simulink model "LunarMicrogrid_Full_Arch"  (R2026b)
settings: Solver=ode23t  StopTime=simulation.timeSim  MaxStep=1/(5*solarPlant.converterSwitchingFrequency)  AbsTol=1e-3
PreLoadFcn:
  | run('LunarMicrogridA_Data');
values from neighbouring files (symbols this model uses):
  Csc = Csc_cell/Ns_sc*Np_sc    (= 200)    [LunarDAB_Params.m]
  eta_sc = 0.95    [LunarDAB_Params.m]
  fsw = 100e3    (= 100000)    [LunarDAB_Params.m]
  k_restore = 1    [LunarDAB_Params.m]
  kiCurrent = 2    [LunarDAB_Params.m]
  kiVoltage = 8    [LunarDAB_Params.m]
  kpCurrent = 0.005    [LunarDAB_Params.m]
  kpVoltage = 0.4    [LunarDAB_Params.m]
  lTotal = lSeries + Llk    [LunarDAB_Params.m]
  P170_dt = 1e-4    (= 0.0001)    [P170_PV_Initialize.m]
  P170_Imp = im(ix)    [P170_PV_Initialize.m]
  P170_Vmp = vm(ix)    [P170_PV_Initialize.m]
  Rd_bat = dV_droop/Ibat_max    (= 0.232258064516)    [LunarDAB_Params.m]
  SC_enable = 1    [LunarDAB_Params.m]
  thetaIC = 0    [LunarDAB_Params.m]
  thetaMaxDab = pi/4    (= 0.785398163397)    [LunarDAB_Params.m]
  Tsw = 1/fsw    (= 1e-05)    [LunarDAB_Params.m]
  Vsc0 = sqrt((Vsc_max^2 + Vsc_min^2)/2)    [LunarDAB_Params.m]
  Vsc_max = 119    [LunarDAB_Params.m]
  Vsc_min = 66    [LunarDAB_Params.m]
undefined symbols (not defined in the file or in its folder): a_lpf_sys, battery, bms, connectedLoad, dcVoltage, DiscIntNeverNeededParam, eta_dab, Ibat_sign, mmc, Ndab, P170_T, pvDroop, sc, sensor, socLimit, solarPlant
libraries: sl_discontinuities x13, fl_lib x13, nesl_utility x13, simulink x7, batteryecm_lib x1, simulink_extras x1, ee_lib x1
(part 4 of 8)

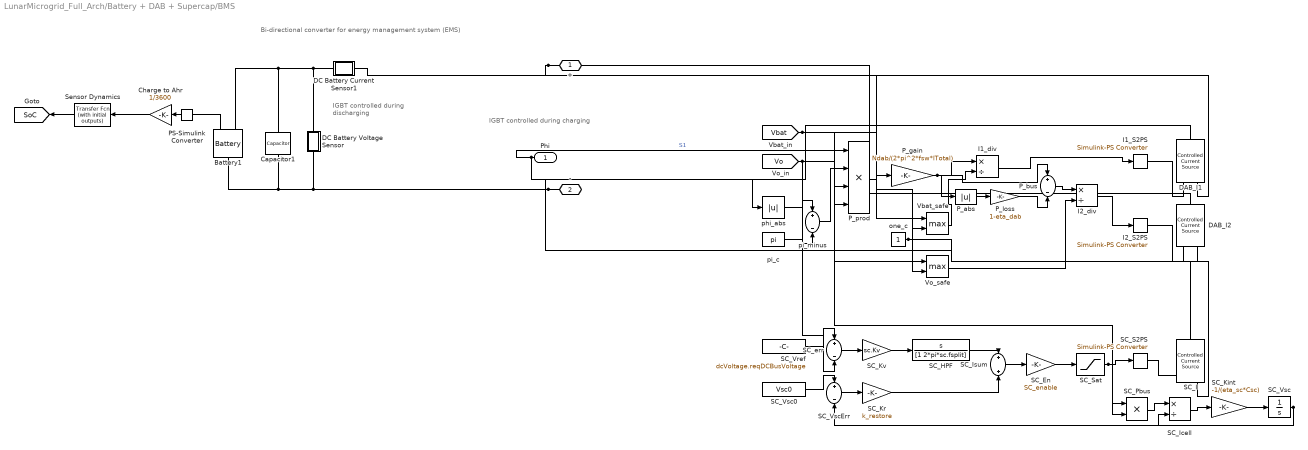
== system LunarMicrogrid_Full_Arch/Battery + DAB + Supercap/BMS ==
  note: IGBT controlled during charging
  note: Bi-directional converter for energy management system (EMS)
  note: IGBT controlled during discharging
  Phi : Inport
  Battery1 : batteryecm_lib/Battery  Vnom=battery.nominalBatteryVoltage V  prm_dir=1  R1_dis=2 Ohm  R1_ch=2 Ohm  R1=0.01 Ohm  prm_AH=2  AH=connectedLoad.batteryAmpHr hr*A  V1=battery.minBatteryNominalVoltage V  AH1=connectedLoad.batteryAmpHr*0.2 hr*A  prm_R2=2  R2=2000 Ohm  Tmeas=298.15 K  charge_measurement_port=simscape.enum.battery.enable.yes  prm_dyn=1  Rp1=0.005 Ohm  tau1=30 s  Rp2=0.005 Ohm  tau2=30 s  Rp3=0.005 Ohm  tau3=30 s  Rp4=0.005 Ohm  tau4=30 s  Rp5=0.005 Ohm  tau5=30 s  prm_fade=1  N_fade=100  AH_fade=45 hr*A  R1_fade=2.02 Ohm  R1_ch_fade=2.02 Ohm  V1_fade=10.35 V  prm_age=1  prm_age_OCV=1  OCV_age=0.9  SOC_age=60  Tmeas_age=298.15 K  delta_time_age_vec=[0] d  temperature_age_vec=[273] K  OCV_scaling_age=2.2134e6  OCV_offset_age=1.632e6  temp_exp_age=0.515833569 V  t_exp_age=0.75  Vnom_T2=12 V  R1_T2=2.2 Ohm  R1_T2_dis=2.2 Ohm  R1_T2_ch=2.2 Ohm  V1_T2=11.4 V  R2_T2=2200 Ohm  Rp1_T2=0.005 Ohm  tau1_T2=30 s  Rp2_T2=0.005 Ohm  tau2_T2=30 s  Rp3_T2=0.005 Ohm  tau3_T2=30 s  Rp4_T2=0.005 Ohm  tau4_T2=30 s  Rp5_T2=0.005 Ohm  tau5_T2=30 s  Tmeas2=273.15 K  thermal_port=simscape.enum.thermaleffects.omit  thermal_mass=30000 J/K  i_specify=off  i_priority=None  i=0 A  i_nominal_specify=off  i_nominal_value=1  i_nominal_unit=A  v_specify=off  v_priority=None  v=0 V  v_nominal_specify=off  v_nominal_value=1  v_nominal_unit=V  charge_specify=on  charge_priority=High  charge=batteryInitialStateOfCharge hr*A  charge_nominal_specify=off  charge_nominal_value=1  charge_nominal_unit=A*hr  num_cycles_specify=off  num_cycles_priority=High  num_cycles=0  num_cycles_nominal_specify=off  num_cycles_nominal_value=1  num_cycles_nominal_unit=1  temperature_specify=off  temperature_priority=High  temperature=298.15 K  temperature_nominal_specify=off  temperature_nominal_value=1  temperature_nominal_unit=K
  Capacitor1 : fl_lib/Electrical/Electrical Elements/Capacitor  c=boost.outputCapacitor F  r=1e-6 Ohm  g=0 1/Ohm  i_specify=off  i_priority=None  i=0 A  i_nominal_specify=off  i_nominal_value=1  i_nominal_unit=A  v_specify=off  v_priority=None  v=0 V  v_nominal_specify=off  v_nominal_value=1  v_nominal_unit=V  vc_specify=on  vc_priority=High  vc=batteryInputCapacitorInitialVoltage V  vc_nominal_specify=off  vc_nominal_value=1  vc_nominal_unit=V
  Charge to Ahr : Gain  Gain=1/3600
  DAB_I1 : fl_lib/Electrical/Electrical Sources/Controlled Current Source
  DAB_I2 : fl_lib/Electrical/Electrical Sources/Controlled Current Source
  DC Battery Current Sensor1 : Subsystem
      mask Display: disp('i');
  DC Battery Voltage Sensor : Subsystem
      mask Display: disp('v');
  I1_S2PS : nesl_utility/Simulink-PS Converter  PhysicalDomain=network_engine_domain  SubClassName=ps_input  LeftPortType=input  RightPortType=output  PseudoPeriodic=off  Frequencies=[]  NoiseDistribution=none  NoiseParameters=[]  Unit=1  AffineConversion=off  FilteringAndDerivatives=provide  SimscapeFilterOrder=1  InputFilterTimeConstant=0.001  UdotUserProvided=0
  I1_div : Product  Inputs=*/
  I2_S2PS : nesl_utility/Simulink-PS Converter  PhysicalDomain=network_engine_domain  SubClassName=ps_input  LeftPortType=input  RightPortType=output  PseudoPeriodic=off  Frequencies=[]  NoiseDistribution=none  NoiseParameters=[]  Unit=1  AffineConversion=off  FilteringAndDerivatives=provide  SimscapeFilterOrder=1  InputFilterTimeConstant=0.001  UdotUserProvided=0
  I2_div : Product  Inputs=*/
  PS-Simulink Converter : nesl_utility/PS-Simulink Converter  PhysicalDomain=network_engine_domain  SubClassName=ps_output  LeftPortType=input  RightPortType=output  PseudoPeriodic=off  Frequencies=[]  VectorFormat=1-D array  Unit=inherit  AffineConversion=off
  P_abs : Abs  SaturateOnIntegerOverflow=off
  P_bus : Sum  Inputs=+-
  P_gain : Gain  Gain=Ndab/(2*pi^2*fsw*lTotal)
  P_loss : Gain  Gain=1-eta_dab
  P_prod : Product  Inputs=4
  SC_En : Gain  Gain=SC_enable
  SC_HPF : TransferFcn  Numerator=[1 0]  Denominator=[1 2*pi*sc.fsplit]
  SC_I : fl_lib/Electrical/Electrical Sources/Controlled Current Source
  SC_Icell : Product  Inputs=*/
  SC_Isum : Sum
  SC_Kint : Gain  Gain=-1/(eta_sc*Csc)
  SC_Kr : Gain  Gain=k_restore
  SC_Kv : Gain  Gain=sc.Kv
  SC_Pbus : Product
  SC_S2PS : nesl_utility/Simulink-PS Converter  PhysicalDomain=network_engine_domain  SubClassName=ps_input  LeftPortType=input  RightPortType=output  PseudoPeriodic=off  Frequencies=[]  NoiseDistribution=none  NoiseParameters=[]  Unit=1  AffineConversion=off  FilteringAndDerivatives=provide  SimscapeFilterOrder=1  InputFilterTimeConstant=0.001  UdotUserProvided=0
  SC_Sat : Saturate  UpperLimit=sc.Imax  LowerLimit=-sc.Imax
  SC_Vref : Constant  Value=dcVoltage.reqDCBusVoltage
  SC_Vsc : Integrator  InitialCondition=Vsc0  LimitOutput=on  UpperSaturationLimit=Vsc_max  LowerSaturationLimit=Vsc_min
  SC_Vsc0 : Constant  Value=Vsc0
  SC_VscErr : Sum  Inputs=+-
  SC_err : Sum  Inputs=+-
  Sensor Dynamics : simulink_extras/Additional Linear/Transfer Fcn (with initial outputs)  N=[1]  D=[1/sensor.samplingFreq 1]  Y0=batteryInitialStateOfCharge  U0=0
  Vbat_safe : MinMax  Function=max  Inputs=2
  Vo_safe : MinMax  Function=max  Inputs=2
  one_c : Constant
  phi_abs : Abs  SaturateOnIntegerOverflow=off
  pi_c : Constant  Value=pi
  pi_minus : Sum  Inputs=+-
  + : PMIOPort  Side=Right
  - : PMIOPort  Port=2  Side=Right
  tag scope: SoC=global
  wires:
  PS-Simulink Converter/1 -> Charge to Ahr/1
  Sensor Dynamics/1 -> [SoC]
  Charge to Ahr/1 -> Sensor Dynamics/1
  Phi/1 -> phi_abs/1, P_prod/1  "S1"
  pi_c/1 -> pi_minus/1
  phi_abs/1 -> pi_minus/2
  pi_minus/1 -> P_prod/2
  [Vbat] -> P_prod/3, Vbat_safe/1
  [Vo] -> P_prod/4, Vo_safe/1, SC_err/2, SC_Pbus/2
  P_prod/1 -> P_gain/1
  one_c/1 -> Vbat_safe/2, Vo_safe/2
  P_gain/1 -> I1_div/1, P_abs/1, P_bus/1
  Vbat_safe/1 -> I1_div/2
  P_abs/1 -> P_loss/1
  P_loss/1 -> P_bus/2
  P_bus/1 -> I2_div/1
  Vo_safe/1 -> I2_div/2
  SC_Vref/1 -> SC_err/1
  SC_err/1 -> SC_Kv/1
  SC_Kv/1 -> SC_HPF/1
  SC_Vsc0/1 -> SC_VscErr/1
  SC_Vsc/1 -> SC_VscErr/2, SC_Icell/2
  SC_VscErr/1 -> SC_Kr/1
  SC_HPF/1 -> SC_Isum/1
  SC_Kr/1 -> SC_Isum/2
  SC_Isum/1 -> SC_En/1
  SC_En/1 -> SC_Sat/1
  SC_Sat/1 -> SC_Pbus/1, SC_S2PS/1
  SC_Pbus/1 -> SC_Icell/1
  SC_Icell/1 -> SC_Kint/1
  SC_Kint/1 -> SC_Vsc/1
  I1_div/1 -> I1_S2PS/1
  I2_div/1 -> I2_S2PS/1
  connections:
  Battery1/RConn1 -- Capacitor1/RConn1 -- DC Battery Voltage Sensor/LConn1 -- DAB_I1/LConn1 -- DAB_I2/RConn2 -- -/RConn1 -- SC_I/RConn2
  Battery1/LConn2 -- PS-Simulink Converter/LConn1
  DC Battery Current Sensor1/LConn1 -- DC Battery Voltage Sensor/RConn1 -- Battery1/LConn1 -- Capacitor1/LConn1
  I1_S2PS/RConn1 -- DAB_I1/RConn1
  I2_S2PS/RConn1 -- DAB_I2/RConn1
  SC_S2PS/RConn1 -- SC_I/RConn1
  DAB_I1/RConn2 -- DC Battery Current Sensor1/RConn1
  +/RConn1 -- DAB_I2/LConn1 -- SC_I/LConn1

== system LunarMicrogrid_Full_Arch/Load (Site A)/Load ==
  AC Current Sensor2 : Subsystem
      mask Display: disp('i');
  Load : Subsystem
  Load Flag : Subsystem
  Load Resistance : fl_lib/Electrical/Electrical Elements/Variable Resistor  Rmin=0 Ohm  thermalEnable=false  thermal_mass=1 J/K  i_specify=off  i_priority=None  i=5 A  i_nominal_specify=off  i_nominal_value=1  i_nominal_unit=A  v_specify=off  v_priority=None  v=0 V  v_nominal_specify=off  v_nominal_value=1  v_nominal_unit=V  T_specify=off  T_priority=None  T=300 K  T_nominal_specify=off  T_nominal_value=1  T_nominal_unit=K
  SPST Switch : ee_lib/Switches & Breakers/SPST Switch  R_closed=0.01 Ohm  G_open=1e-6 S  Threshold=0.5 V  Width=0 V  model_dynamics=0  t_on=1e-3 s  t_off=1e-3 s  initial_vT=0 V
  + : PMIOPort  Side=Left
  - : PMIOPort  Port=2  Side=Right
  connections:
  +/RConn1 -- SPST Switch/LConn2
  Load Resistance/LConn2 -- AC Current Sensor2/LConn1
  Load Resistance/RConn1 -- -/RConn1
  Load/RConn1 -- Load Resistance/LConn1
  Load Flag/RConn1 -- SPST Switch/LConn1
  AC Current Sensor2/RConn1 -- SPST Switch/RConn1

== system LunarMicrogrid_Full_Arch/Low Voltage Bus (120 V)/DC Output Voltage Sensor ==
  PS-Simulink Converter : nesl_utility/PS-Simulink Converter  PhysicalDomain=network_engine_domain  SubClassName=ps_output  LeftPortType=input  RightPortType=output  PseudoPeriodic=off  Frequencies=[]  VectorFormat=1-D array  Unit=1  AffineConversion=off
  Sensor dynamics : TransferFcn  Numerator=1  Denominator=[1/sensor.samplingFreq 1]
  Voltage Sensor : fl_lib/Electrical/Electrical Sensors/Voltage Sensor
  - : PMIOPort  Side=Left
  + : PMIOPort  Port=2  Side=Right
  tag scope: Vo=global
  wires:
  PS-Simulink Converter/1 -> Sensor dynamics/1
  Sensor dynamics/1 -> [Vo]
  connections:
  Voltage Sensor/RConn2 -- -/RConn1
  Voltage Sensor/RConn1 -- PS-Simulink Converter/LConn1
  Voltage Sensor/LConn1 -- +/RConn1

== system LunarMicrogrid_Full_Arch/Monitoring/PV System Monitoring Panel ==
  note: Red - Overload , reduce the load and manually toggle the switch to restart the system
  note: Solar PV System Monitoring Panel
  note: Simulation time:
      | Increase the value for 'simulation.timeSim' to simulate for longer when exploring mode changes.
  note: Inputs:
      | Use the rotary controls to change the irradiance and load resistance during simulation.
  note: System overload (Mode-6):
      | System overload is triggered 'olTime' sec after the overload event. This delay is to ensure that it is not triggered because of transients. Parameter 'olTime' can be modified in the supporting livescript.
  note: Efficiency:
      | Percent efficiency may exceed 100% due to the stored energy in the inductor and capacitor. Efficiency value will be accurate in steady state.
  note: Battery sign convention:
      | +ve value for charging
      | -ve value for discharging
  Display{,1..6} (7 alike) : DisplayBlock  Transparency=1  GridColor=[0.502, 0.502, 0.502]
  Half Gauge : SemiCircularGaugeBlock  ScaleMin=20  FontColor=[0.0, 0.0, 0.0]
  Half Gauge1 : SemiCircularGaugeBlock  FontColor=[0.0, 0.0, 0.0]
  Lamp : LampBlock  DefaultColor=[192.0, 192.0, 192.0]
  Linear Gauge : LinearGaugeBlock  ScaleMin=-100  FontColor=[0.0, 0.0, 0.0]
  Monitoring : Subsystem
  PV MPPT Battery Charge Load ShutDown : LampBlock  DefaultColor=[192.0, 192.0, 192.0]
  PV MPPT Battery Discharge : LampBlock  DefaultColor=[192.0, 192.0, 192.0]
  PV MPPT Battery charge : LampBlock  DefaultColor=[192.0, 192.0, 192.0]
  PV ShutDown Battery Discharge : LampBlock  DefaultColor=[192.0, 192.0, 192.0]
  PV ShutDown Battery Isolated System ShutDown : LampBlock  DefaultColor=[192.0, 192.0, 192.0]
  PV Volt Control Battery Isolated : LampBlock  DefaultColor=[192.0, 192.0, 192.0]
  Start Mode : LampBlock  DefaultColor=[192.0, 192.0, 192.0]
  Toggle Switch1 : ToggleSwitchBlock

== system LunarMicrogrid_Full_Arch/PV Array + Converter/Irradiance ==
  Goto11 : Terminator
  Profile : FromWorkspace  VariableName=G_sim  Interpolate=off  OutputAfterFinalValue=Holding final value
  Sensor dynamics : TransferFcn  Numerator=1  Denominator=[1/sensor.samplingFreq 1]
  Solar Irradiance W/m2 : Gain
  Irad : Outport
  wires:
  Solar Irradiance W/m2/1 -> Irad/1, Sensor dynamics/1
  Profile/1 -> Solar Irradiance W/m2/1
  Sensor dynamics/1 -> Goto11/1

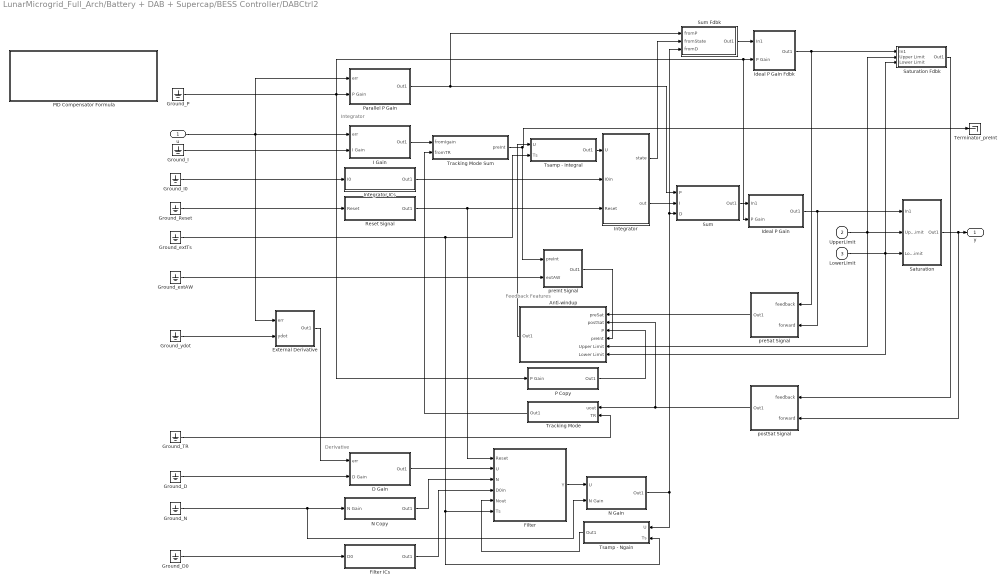
== system LunarMicrogrid_Full_Arch/Battery + DAB + Supercap/BESS Controller/DABCtrl2 ==
  note: Feedback Features
  note: Derivative
  note: Integrator
  u : Inport  SampleTime=SampleTime
  UpperLimit : Inport  Port=2
  LowerLimit : Inport  Port=3
  Anti-windup : Subsystem  Variant=on  VariantControlMode=label  VariantControl=Variant1  LabelModeActiveChoice=DiscClampingParallel
  D Gain : Subsystem  Variant=on  VariantControlMode=label  VariantControl=Variant1  LabelModeActiveChoice=Disabled
  External Derivative : Subsystem  Variant=on  VariantControlMode=label  VariantControl=Variant1  LabelModeActiveChoice=Disabled
  Filter : Subsystem  Variant=on  VariantControlMode=label  LabelModeActiveChoice=Disabled
  Filter ICs : Subsystem  Variant=on  VariantControlMode=label  VariantControl=Variant1  LabelModeActiveChoice=Disabled
  Ground_D : Ground
  Ground_D0 : Ground
  Ground_I : Ground
  Ground_I0 : Ground
  Ground_N : Ground
  Ground_P : Ground
  Ground_Reset : Ground
  Ground_TR : Ground  DisableCoverage=on
  Ground_extAW : Ground
  Ground_extTs : Ground
  Ground_ydot : Ground
  I Gain : Subsystem  Variant=on  VariantControlMode=label  VariantControl=Variant1  LabelModeActiveChoice=InternalParameters
  Ideal P Gain : Subsystem  Variant=on  VariantControlMode=label  VariantControl=Variant1  LabelModeActiveChoice=Disabled
  Ideal P Gain Fdbk : Subsystem  Variant=on  VariantControlMode=label  VariantControl=Variant1  LabelModeActiveChoice=Disabled
  Integrator : Subsystem  Variant=on  VariantControlMode=label  LabelModeActiveChoice=Discrete
  Integrator ICs : Subsystem  Variant=on  VariantControlMode=label  VariantControl=Variant1  LabelModeActiveChoice=InternalICs
  N Copy : Subsystem  Variant=on  VariantControlMode=label  LabelModeActiveChoice=Disabled_SignalSpec
  N Gain : Subsystem  Variant=on  VariantControlMode=label  VariantControl=Variant1  LabelModeActiveChoice=Disabled
  P Copy : Subsystem  Variant=on  VariantControlMode=label  LabelModeActiveChoice=Disabled
  PID Compensator Formula : Subsystem
      mask Display: image('/MATLAB/toolbox/simulink/library/pid/pid_Images/PI_Parallel_DT_0.png','center');
  Parallel P Gain : Subsystem  Variant=on  VariantControlMode=label  VariantControl=Variant1  LabelModeActiveChoice=InternalParameters
  Reset Signal : Subsystem  Variant=on  VariantControlMode=label  VariantControl=Variant1  LabelModeActiveChoice=Disabled
  Saturation : Subsystem  Variant=on  VariantControlMode=label  LabelModeActiveChoice=External
  Saturation Fdbk : Subsystem  Variant=on  VariantControlMode=label  LabelModeActiveChoice=Disabled
  Sum : Subsystem  Variant=on  VariantControlMode=label  LabelModeActiveChoice=Sum_PI
  Sum Fdbk : Subsystem  DisableCoverage=on  Variant=on  VariantControlMode=label  LabelModeActiveChoice=Disabled
  Terminator_preInt : Terminator
  Tracking Mode : Subsystem  Variant=on  VariantControlMode=label  VariantControl=Variant1  LabelModeActiveChoice=Disabled
  Tracking Mode Sum : Subsystem  Variant=on  VariantControlMode=label  LabelModeActiveChoice=Passthrough
  Tsamp - Integral : Subsystem  Variant=on  VariantControlMode=label  LabelModeActiveChoice=Disabled_SignalSpec
  Tsamp - Ngain : Subsystem  Variant=on  VariantControlMode=label  LabelModeActiveChoice=Passthrough
  postSat Signal : Subsystem  Variant=on  VariantControlMode=label  VariantControl=Variant1  LabelModeActiveChoice=Forward
  preInt Signal : Subsystem  Variant=on  VariantControlMode=label  VariantControl=Variant1  LabelModeActiveChoice=InternalPreInt
  preSat Signal : Subsystem  Variant=on  VariantControlMode=label  VariantControl=Variant1  LabelModeActiveChoice=Forward
  y : Outport  SampleTime=SampleTime
  wires:
  Ground_extAW/1 -> preInt Signal/2(extAW)
  preInt Signal/1(Out1) -> Anti-windup/4(preInt)
  External Derivative/1(Out1) -> D Gain/1(err)
  Ground_ydot/1 -> External Derivative/2(ydot)
  LowerLimit/1 -> Saturation/3(Lower Limit), Anti-windup/6(Lower Limit), Saturation Fdbk/3(Lower Limit)
  UpperLimit/1 -> Saturation/2(Upper Limit), Saturation Fdbk/2(Upper Limit), Anti-windup/5(Upper Limit)
  Tsamp - Ngain/1(Out1) -> Filter/5(Nout)
  Anti-windup/1(Out1) -> Tsamp - Integral/1(U)
  Ground_extTs/1 -> Tsamp - Integral/2(Ts), Filter/6(Ts), Tsamp - Ngain/2(Ts)
  Tsamp - Integral/1(Out1) -> Integrator/1(U)
  Tracking Mode/1(Out1) -> Tracking Mode Sum/2(fromTR)
  Ground_I0/1 -> Integrator ICs/1(I0)
  Filter ICs/1(Out1) -> Filter/4(D0in)
  N Copy/1(Out1) -> Filter/3(N)
  D Gain/1(Out1) -> Filter/2(U)
  Ground_D0/1 -> Filter ICs/1(D0)
  Ground_Reset/1 -> Reset Signal/1(Reset)
  N Gain/1(Out1) -> Tsamp - Ngain/1(U), Sum/3(D), Sum Fdbk/3(fromD)
  postSat Signal/1(Out1) -> Anti-windup/2(postSat), Tracking Mode/1(uout)
  preSat Signal/1(Out1) -> Anti-windup/1(preSat)
  Saturation Fdbk/1(Out1) -> postSat Signal/1(feedback)
  P Copy/1(Out1) -> Anti-windup/3(P)
  Ground_TR/1 -> Tracking Mode/2(TR)
  Ground_N/1 -> N Copy/1(N Gain), N Gain/2(N Gain)
  Ideal P Gain Fdbk/1(Out1) -> preSat Signal/1(feedback), Saturation Fdbk/1(In1)
  Sum Fdbk/1(Out1) -> Ideal P Gain Fdbk/1(In1)
  I Gain/1(Out1) -> Tracking Mode Sum/1(fromIgain)
  Saturation/1(Out1) -> y/1, postSat Signal/2(forward)
  Filter/1(Y) -> N Gain/1(U)
  Ground_D/1 -> D Gain/2(D Gain)
  Ideal P Gain/1(Out1) -> Saturation/1(In1), preSat Signal/2(forward)
  u/1 -> External Derivative/1(err), Parallel P Gain/1(err), I Gain/1(err)
  Parallel P Gain/1(Out1) -> Sum/1(P), Sum Fdbk/1(fromP)
  Sum/1(Out1) -> Ideal P Gain/1(In1)
  Ground_P/1 -> Ideal P Gain Fdbk/2(P Gain), Ideal P Gain/2(P Gain), Parallel P Gain/2(P Gain), P Copy/1(P Gain)
  Tracking Mode Sum/1(preInt) -> Terminator_preInt/1, preInt Signal/1(preInt)
  Ground_I/1 -> I Gain/2(I Gain)
  Integrator ICs/1(Out1) -> Integrator/2(I0in)
  Integrator/2(out) -> Sum/2(I)
  Integrator/1(state) -> Sum Fdbk/2(fromState)
  Reset Signal/1(Out1) -> Filter/1(Reset), Integrator/3(Reset)

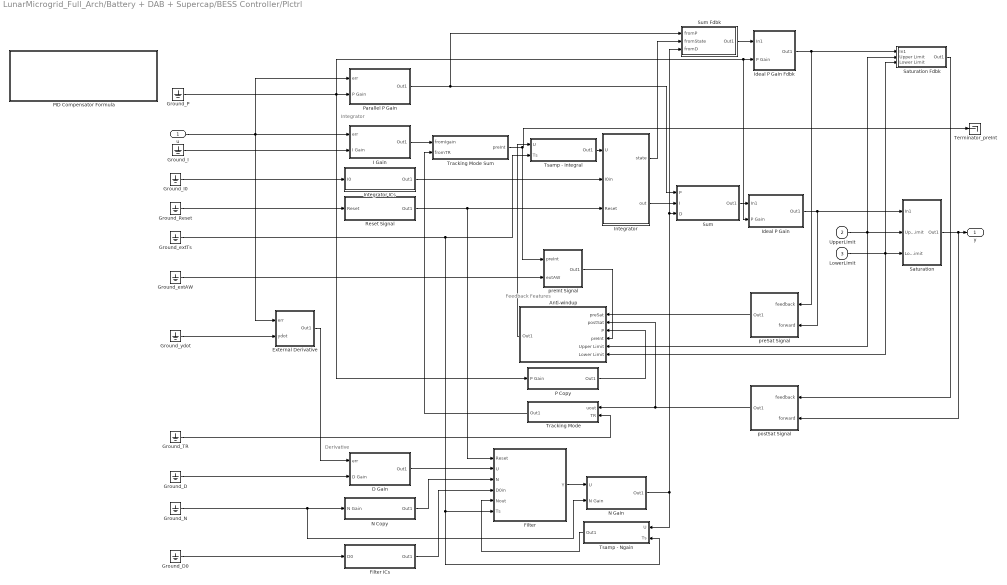
== system LunarMicrogrid_Full_Arch/Battery + DAB + Supercap/BESS Controller/PIctrl ==
  note: Feedback Features
  note: Derivative
  note: Integrator
  u : Inport  SampleTime=SampleTime
  UpperLimit : Inport  Port=2
  LowerLimit : Inport  Port=3
  Anti-windup : Subsystem  Variant=on  VariantControlMode=label  VariantControl=Variant1  LabelModeActiveChoice=DiscClampingParallel
  D Gain : Subsystem  Variant=on  VariantControlMode=label  VariantControl=Variant1  LabelModeActiveChoice=Disabled
  External Derivative : Subsystem  Variant=on  VariantControlMode=label  VariantControl=Variant1  LabelModeActiveChoice=Disabled
  Filter : Subsystem  Variant=on  VariantControlMode=label  LabelModeActiveChoice=Disabled
  Filter ICs : Subsystem  Variant=on  VariantControlMode=label  VariantControl=Variant1  LabelModeActiveChoice=Disabled
  Ground_D : Ground
  Ground_D0 : Ground
  Ground_I : Ground
  Ground_I0 : Ground
  Ground_N : Ground
  Ground_P : Ground
  Ground_Reset : Ground
  Ground_TR : Ground  DisableCoverage=on
  Ground_extAW : Ground
  Ground_extTs : Ground
  Ground_ydot : Ground
  I Gain : Subsystem  Variant=on  VariantControlMode=label  VariantControl=Variant1  LabelModeActiveChoice=InternalParameters
  Ideal P Gain : Subsystem  Variant=on  VariantControlMode=label  VariantControl=Variant1  LabelModeActiveChoice=Disabled
  Ideal P Gain Fdbk : Subsystem  Variant=on  VariantControlMode=label  VariantControl=Variant1  LabelModeActiveChoice=Disabled
  Integrator : Subsystem  Variant=on  VariantControlMode=label  LabelModeActiveChoice=Discrete
  Integrator ICs : Subsystem  Variant=on  VariantControlMode=label  VariantControl=Variant1  LabelModeActiveChoice=InternalICs
  N Copy : Subsystem  Variant=on  VariantControlMode=label  LabelModeActiveChoice=Disabled_SignalSpec
  N Gain : Subsystem  Variant=on  VariantControlMode=label  VariantControl=Variant1  LabelModeActiveChoice=Disabled
  P Copy : Subsystem  Variant=on  VariantControlMode=label  LabelModeActiveChoice=Disabled
  PID Compensator Formula : Subsystem
      mask Display: image('/MATLAB/toolbox/simulink/library/pid/pid_Images/PI_Parallel_DT_0.png','center');
  Parallel P Gain : Subsystem  Variant=on  VariantControlMode=label  VariantControl=Variant1  LabelModeActiveChoice=InternalParameters
  Reset Signal : Subsystem  Variant=on  VariantControlMode=label  VariantControl=Variant1  LabelModeActiveChoice=Disabled
  Saturation : Subsystem  Variant=on  VariantControlMode=label  LabelModeActiveChoice=External
  Saturation Fdbk : Subsystem  Variant=on  VariantControlMode=label  LabelModeActiveChoice=Disabled
  Sum : Subsystem  Variant=on  VariantControlMode=label  LabelModeActiveChoice=Sum_PI
  Sum Fdbk : Subsystem  DisableCoverage=on  Variant=on  VariantControlMode=label  LabelModeActiveChoice=Disabled
  Terminator_preInt : Terminator
  Tracking Mode : Subsystem  Variant=on  VariantControlMode=label  VariantControl=Variant1  LabelModeActiveChoice=Disabled
  Tracking Mode Sum : Subsystem  Variant=on  VariantControlMode=label  LabelModeActiveChoice=Passthrough
  Tsamp - Integral : Subsystem  Variant=on  VariantControlMode=label  LabelModeActiveChoice=Disabled_SignalSpec
  Tsamp - Ngain : Subsystem  Variant=on  VariantControlMode=label  LabelModeActiveChoice=Passthrough
  postSat Signal : Subsystem  Variant=on  VariantControlMode=label  VariantControl=Variant1  LabelModeActiveChoice=Forward
  preInt Signal : Subsystem  Variant=on  VariantControlMode=label  VariantControl=Variant1  LabelModeActiveChoice=InternalPreInt
  preSat Signal : Subsystem  Variant=on  VariantControlMode=label  VariantControl=Variant1  LabelModeActiveChoice=Forward
  y : Outport  SampleTime=SampleTime
  wires:
  Ground_extAW/1 -> preInt Signal/2(extAW)
  preInt Signal/1(Out1) -> Anti-windup/4(preInt)
  External Derivative/1(Out1) -> D Gain/1(err)
  Ground_ydot/1 -> External Derivative/2(ydot)
  LowerLimit/1 -> Saturation/3(Lower Limit), Anti-windup/6(Lower Limit), Saturation Fdbk/3(Lower Limit)
  UpperLimit/1 -> Saturation/2(Upper Limit), Saturation Fdbk/2(Upper Limit), Anti-windup/5(Upper Limit)
  Tsamp - Ngain/1(Out1) -> Filter/5(Nout)
  Anti-windup/1(Out1) -> Tsamp - Integral/1(U)
  Ground_extTs/1 -> Tsamp - Integral/2(Ts), Filter/6(Ts), Tsamp - Ngain/2(Ts)
  Tsamp - Integral/1(Out1) -> Integrator/1(U)
  Tracking Mode/1(Out1) -> Tracking Mode Sum/2(fromTR)
  Ground_I0/1 -> Integrator ICs/1(I0)
  Filter ICs/1(Out1) -> Filter/4(D0in)
  N Copy/1(Out1) -> Filter/3(N)
  D Gain/1(Out1) -> Filter/2(U)
  Ground_D0/1 -> Filter ICs/1(D0)
  Ground_Reset/1 -> Reset Signal/1(Reset)
  N Gain/1(Out1) -> Tsamp - Ngain/1(U), Sum/3(D), Sum Fdbk/3(fromD)
  postSat Signal/1(Out1) -> Anti-windup/2(postSat), Tracking Mode/1(uout)
  preSat Signal/1(Out1) -> Anti-windup/1(preSat)
  Saturation Fdbk/1(Out1) -> postSat Signal/1(feedback)
  P Copy/1(Out1) -> Anti-windup/3(P)
  Ground_TR/1 -> Tracking Mode/2(TR)
  Ground_N/1 -> N Copy/1(N Gain), N Gain/2(N Gain)
  Ideal P Gain Fdbk/1(Out1) -> preSat Signal/1(feedback), Saturation Fdbk/1(In1)
  Sum Fdbk/1(Out1) -> Ideal P Gain Fdbk/1(In1)
  I Gain/1(Out1) -> Tracking Mode Sum/1(fromIgain)
  Saturation/1(Out1) -> y/1, postSat Signal/2(forward)
  Filter/1(Y) -> N Gain/1(U)
  Ground_D/1 -> D Gain/2(D Gain)
  Ideal P Gain/1(Out1) -> Saturation/1(In1), preSat Signal/2(forward)
  u/1 -> External Derivative/1(err), Parallel P Gain/1(err), I Gain/1(err)
  Parallel P Gain/1(Out1) -> Sum/1(P), Sum Fdbk/1(fromP)
  Sum/1(Out1) -> Ideal P Gain/1(In1)
  Ground_P/1 -> Ideal P Gain Fdbk/2(P Gain), Ideal P Gain/2(P Gain), Parallel P Gain/2(P Gain), P Copy/1(P Gain)
  Tracking Mode Sum/1(preInt) -> Terminator_preInt/1, preInt Signal/1(preInt)
  Ground_I/1 -> I Gain/2(I Gain)
  Integrator ICs/1(Out1) -> Integrator/2(I0in)
  Integrator/2(out) -> Sum/2(I)
  Integrator/1(state) -> Sum Fdbk/2(fromState)
  Reset Signal/1(Out1) -> Filter/1(Reset), Integrator/3(Reset)

== system LunarMicrogrid_Full_Arch/Battery + DAB + Supercap/BMS/DC Battery Current Sensor1 ==
  Current Sensor : fl_lib/Electrical/Electrical Sensors/Current Sensor
  PS-Simulink Converter : nesl_utility/PS-Simulink Converter  PhysicalDomain=network_engine_domain  SubClassName=ps_output  LeftPortType=input  RightPortType=output  PseudoPeriodic=off  Frequencies=[]  VectorFormat=1-D array  Unit=1  AffineConversion=off
  Sensor dynamics : TransferFcn  Numerator=1  Denominator=[1/sensor.samplingFreq 1]
  - : PMIOPort  Side=Left
  + : PMIOPort  Port=2  Side=Right
  tag scope: Ibattery=global
  wires:
  PS-Simulink Converter/1 -> Sensor dynamics/1
  Sensor dynamics/1 -> [Ibattery]
  connections:
  Current Sensor/RConn1 -- PS-Simulink Converter/LConn1
  +/RConn1 -- Current Sensor/LConn1
  Current Sensor/RConn2 -- -/RConn1

== system LunarMicrogrid_Full_Arch/Battery + DAB + Supercap/BMS/DC Battery Voltage Sensor ==
  PS-Simulink Converter : nesl_utility/PS-Simulink Converter  PhysicalDomain=network_engine_domain  SubClassName=ps_output  LeftPortType=input  RightPortType=output  PseudoPeriodic=off  Frequencies=[]  VectorFormat=1-D array  Unit=1  AffineConversion=off
  Sensor dynamics : TransferFcn  Numerator=1  Denominator=[1/sensor.samplingFreq 1]
  Voltage Sensor : fl_lib/Electrical/Electrical Sensors/Voltage Sensor
      settings: LogSimulationData=on
  - : PMIOPort  Side=Left
  + : PMIOPort  Port=2  Side=Right
  tag scope: Vbat=global
  wires:
  PS-Simulink Converter/1 -> Sensor dynamics/1
  Sensor dynamics/1 -> [Vbat]
  connections:
  Voltage Sensor/LConn1 -- +/RConn1
  Voltage Sensor/RConn1 -- PS-Simulink Converter/LConn1
  Voltage Sensor/RConn2 -- -/RConn1

== system LunarMicrogrid_Full_Arch/Load (Site A)/Load/AC Current Sensor2 ==
  Current Sensor : fl_lib/Electrical/Electrical Sensors/Current Sensor
  PS-Simulink Converter : nesl_utility/PS-Simulink Converter  PhysicalDomain=network_engine_domain  SubClassName=ps_output  LeftPortType=input  RightPortType=output  PseudoPeriodic=off  Frequencies=[]  VectorFormat=1-D array  Unit=1  AffineConversion=off
  Scope : Scope
      settings: ActiveDisplayYMinimum=-2.69141  ActiveDisplayYMaximum=24.19807  DataLoggingVariableName=ScopeData4
  Sensor dynamics : TransferFcn  Numerator=1  Denominator=[1/sensor.samplingFreq 1]
  - : PMIOPort  Side=Left
  + : PMIOPort  Port=2  Side=Right
  tag scope: Iload=global
  wires:
  PS-Simulink Converter/1 -> Sensor dynamics/1
  Sensor dynamics/1 -> Scope/1, [Iload]
  connections:
  Current Sensor/RConn1 -- PS-Simulink Converter/LConn1
  +/RConn1 -- Current Sensor/LConn1
  Current Sensor/RConn2 -- -/RConn1

== system LunarMicrogrid_Full_Arch/Load (Site A)/Load/Load ==
  " 1" : Constant  Value=1e-3
  " 2" : Constant  Value=dcVoltage.reqDCBusVoltage*dcVoltage.reqDCBusVoltage*1e-3
  Divide : Product  Inputs=*/
  Load Power (kW) : Gain
  Profile : FromWorkspace  VariableName=Pload_local_sim  Interpolate=off  OutputAfterFinalValue=Holding final value
  Simulink-PS Converter1 : nesl_utility/Simulink-PS Converter  PhysicalDomain=network_engine_domain  SubClassName=ps_input  LeftPortType=input  RightPortType=output  PseudoPeriodic=off  Frequencies=[]  NoiseDistribution=none  NoiseParameters=[]  Unit=1  AffineConversion=off  FilteringAndDerivatives=filter  SimscapeFilterOrder=1  InputFilterTimeConstant=1e-3  UdotUserProvided=0
  Switch : Switch  Criteria=u2 > Threshold  SaturateOnIntegerOverflow=off  InputSameDT=off
  R : PMIOPort  Side=Right
  wires:
  Load Power (kW)/1 -> Switch/1, Switch/2
  " 1"/1 -> Switch/3
  " 2"/1 -> Divide/1
  Switch/1 -> Divide/2
  Divide/1 -> Simulink-PS Converter1/1
  Profile/1 -> Load Power (kW)/1
  connections:
  Simulink-PS Converter1/RConn1 -- R/RConn1

== system LunarMicrogrid_Full_Arch/Load (Site A)/Load/Load Flag ==
  Data Type Conversion1 : DataTypeConversion  SaturateOnIntegerOverflow=off  RndMeth=Floor
  NOT : Logic  Operator=NOT  IconShape=distinctive  AllPortsSameDT=off  OutDataTypeStr=boolean
  OR : Logic  Operator=OR  IconShape=distinctive  AllPortsSameDT=off  OutDataTypeStr=boolean
  Simulink-PS Converter2 : nesl_utility/Simulink-PS Converter  PhysicalDomain=network_engine_domain  SubClassName=ps_input  LeftPortType=input  RightPortType=output  PseudoPeriodic=off  Frequencies=[]  NoiseDistribution=none  NoiseParameters=[]  Unit=1  AffineConversion=off  FilteringAndDerivatives=provide  SimscapeFilterOrder=1  InputFilterTimeConstant=0.001  UdotUserProvided=0
  CB : PMIOPort  Side=Right
  wires:
  [loadShutDown] -> OR/1
  Data Type Conversion1/1 -> Simulink-PS Converter2/1
  [ShutDown] -> OR/2  "System Status"
  OR/1 -> NOT/1
  NOT/1 -> Data Type Conversion1/1
  connections:
  Simulink-PS Converter2/RConn1 -- CB/RConn1

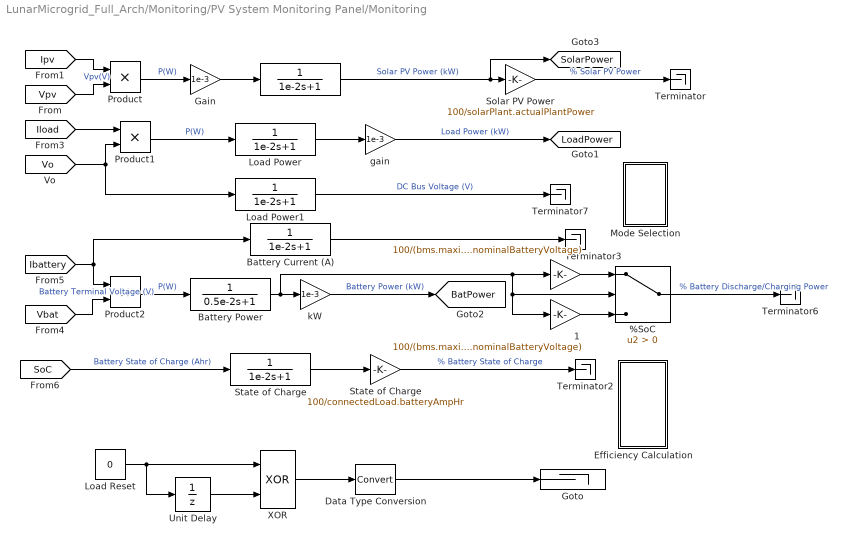
== system LunarMicrogrid_Full_Arch/Monitoring/PV System Monitoring Panel/Monitoring ==
  " " : Gain  Gain=100/(bms.maximumChargingCurrentLimit*battery.nominalBatteryVoltage)
  "  " : TransferFcn  Denominator=[1e-2 1]
  " 1" : Gain  Gain=100/(bms.maximumDisChargingCurrent*battery.nominalBatteryVoltage)
  " State of Charge" : Gain  Gain=100/connectedLoad.batteryAmpHr
  %SoC : Switch  Criteria=u2 > Threshold  SaturateOnIntegerOverflow=off  InputSameDT=off
  Battery Current (A) : TransferFcn  Denominator=[1e-2 1]
  Battery Power : TransferFcn  Denominator=[0.5e-2 1]
  Data Type Conversion : DataTypeConversion  SaturateOnIntegerOverflow=off  RndMeth=Floor
  Efficiency Calculation : Subsystem
  Gain : Gain  Gain=1e-3
  Goto : Terminator
  Load Power : TransferFcn  Denominator=[1e-2 1]
  Load Power1 : TransferFcn  Denominator=[1e-2 1]
  Load Reset : Constant  Value=0
  Mode Selection : Subsystem
  Product : Product
  Product1 : Product
  Product2 : Product
  Solar PV Power : Gain  Gain=100/solarPlant.actualPlantPower
  State of Charge : TransferFcn  Denominator=[1e-2 1]
  Terminator{,2..3,6..7} (5 alike) : Terminator
  Unit Delay : UnitDelay  SampleTime=1e-3
  XOR : Logic  Operator=XOR  IconShape=distinctive  AllPortsSameDT=off  OutDataTypeStr=boolean
  gain : Gain  Gain=1e-3
  kW : Gain  Gain=1e-3
  tag scope: BatPower=global, LoadPower=global, SolarPower=global
  wires:
  [Vpv] -> Product/2  "Vpv(V)"
  Load Power/1 -> gain/1
  Product1/1 -> Load Power/1  "P(W)"
  [Vbat] -> Product2/2  "Battery Terminal Voltage (V)"
  [Iload] -> Product1/1
  Battery Power/1 -> kW/1, " 1"/1, %SoC/2, " "/1
  "  "/1 -> [SolarPower], Solar PV Power/1  "Solar PV Power (kW)"
  [Ibattery] -> Product2/1, Battery Current (A)/1
  Product2/1 -> Battery Power/1  "P(W)"
  [Ipv] -> Product/1
  [Vo] -> Product1/2, Load Power1/1
  Product/1 -> Gain/1  "P(W)"
  [SoC] -> State of Charge/1  "Battery State of Charge (Ahr)"
  Solar PV Power/1 -> Terminator/1  "% Solar PV Power"
  gain/1 -> [LoadPower]  "Load Power (kW)"
  kW/1 -> [BatPower]  "Battery Power (kW)"
  State of Charge/1 -> " State of Charge"/1
  " State of Charge"/1 -> Terminator2/1  "% Battery State of Charge"
  " "/1 -> %SoC/1
  " 1"/1 -> %SoC/3
  %SoC/1 -> Terminator6/1  "% Battery Discharge/Charging Power"
  Battery Current (A)/1 -> Terminator3/1
  Gain/1 -> "  "/1
  Load Power1/1 -> Terminator7/1  "DC Bus Voltage (V)"
  XOR/1 -> Data Type Conversion/1
  Load Reset/1 -> XOR/1, Unit Delay/1
  Unit Delay/1 -> XOR/2
  Data Type Conversion/1 -> Goto/1

== system LunarMicrogrid_Full_Arch/Battery + DAB + Supercap/BESS Controller/DABCtrl2/Anti-windup ==
  preSat : Inport  SampleTime=SampleTime
  postSat : Inport  Port=2  SampleTime=SampleTime
  P : Inport  Port=3  SampleTime=SampleTime
  preInt : Inport  Port=4  SampleTime=SampleTime
  Upper Limit : Inport  Port=5  SampleTime=SampleTime
  Lower Limit : Inport  Port=6  SampleTime=SampleTime
  Back Calculation : Subsystem  VariantControl=BackCalculation
  Cont. Clamping Ideal : Subsystem  VariantControl=ContClampingIdeal
  Cont. Clamping Parallel : Subsystem  VariantControl=ContClampingParallel
  Disabled : Subsystem  VariantControl=Disabled
  Disc. Clamping Ideal : Subsystem  VariantControl=DiscClampingIdeal
  Disc. Clamping Parallel : Subsystem  VariantControl=DiscClampingParallel
  Passthrough : Subsystem  VariantControl=Passthrough
  Out1 : Outport  SampleTime=SampleTime

== system LunarMicrogrid_Full_Arch/Battery + DAB + Supercap/BESS Controller/DABCtrl2/D Gain ==
  err : Inport  SampleTime=SampleTime
  D Gain : Inport  Port=2  SampleTime=SampleTime
  Disabled : Subsystem  VariantControl=Disabled
  External Parameters : Subsystem  VariantControl=ExternalParameters
  Internal Parameters : Subsystem  VariantControl=InternalParameters
  Out1 : Outport  SampleTime=SampleTime

== system LunarMicrogrid_Full_Arch/Battery + DAB + Supercap/BESS Controller/DABCtrl2/External Derivative ==
  err : Inport  SampleTime=SampleTime
  ydot : Inport  Port=2  SampleTime=SampleTime
  Disabled : Subsystem  VariantControl=Disabled
  Error : Subsystem  VariantControl=ErrorSignal
  External Ydot : Subsystem  VariantControl=ExternalYdot
  Out1 : Outport  SampleTime=SampleTime

== system LunarMicrogrid_Full_Arch/Battery + DAB + Supercap/BESS Controller/DABCtrl2/Filter ==
  Reset : Inport  SampleTime=SampleTime
  U : Inport  Port=2  SampleTime=SampleTime
  N : Inport  Port=3  SampleTime=SampleTime
  D0in : Inport  Port=4  SampleTime=SampleTime
  Nout : Inport  Port=5  SampleTime=SampleTime
  Ts : Inport  Port=6  SampleTime=SampleTime
  Cont. Filter : Subsystem  VariantControl=ContFilter
  Cont. Filter Only : Subsystem  VariantControl=ContFilterOnly
  Differentiator : Subsystem  VariantControl=Differentiator
  Disabled : Subsystem  VariantControl=Disabled
  Disc. Backward Euler Filter : Subsystem  VariantControl=BackwardEulerFilter
  Disc. Backward Euler Filter Only : Subsystem  VariantControl=BackwardEulerFilterOnly
  Disc. Forward Euler Filter : Subsystem  VariantControl=ForwardEulerFilter
  Disc. Forward Euler Filter Only : Subsystem  VariantControl=ForwardEulerFilterOnly
  Disc. Trapezoidal Filter : Subsystem  VariantControl=TrapezoidalFilter
  Disc. Trapezoidal Filter Only : Subsystem  VariantControl=TrapezoidalFilterOnly
  Passthrough : Subsystem  VariantControl=Passthrough
  Y : Outport  SampleTime=SampleTime

== system LunarMicrogrid_Full_Arch/Battery + DAB + Supercap/BESS Controller/DABCtrl2/Filter ICs ==
  D0 : Inport  SampleTime=SampleTime
  Disabled : Subsystem  VariantControl=Disabled
  External IC : Subsystem  VariantControl=ExternalICs
  Internal IC - Differentiator : Subsystem  VariantControl=InternalICsDifferentiator
  Internal IC - Filter : Subsystem  VariantControl=InternalICsFilter
  Out1 : Outport  SampleTime=SampleTime

== system LunarMicrogrid_Full_Arch/Battery + DAB + Supercap/BESS Controller/DABCtrl2/I Gain ==
  err : Inport  SampleTime=SampleTime
  I Gain : Inport  Port=2  SampleTime=SampleTime
  Disabled : Subsystem  VariantControl=Disabled
  External Parameters : Subsystem  VariantControl=ExternalParameters
  Internal Parameters : Subsystem  VariantControl=InternalParameters
  Out1 : Outport  SampleTime=SampleTime

== system LunarMicrogrid_Full_Arch/Battery + DAB + Supercap/BESS Controller/DABCtrl2/Ideal P Gain ==
  In1 : Inport  SampleTime=SampleTime
  P Gain : Inport  Port=2  SampleTime=SampleTime
  External Parameters : Subsystem  VariantControl=ExternalParameters
  Internal Parameters : Subsystem  VariantControl=InternalParameters
  Passthrough : Subsystem  VariantControl=Disabled
  Out1 : Outport  SampleTime=SampleTime

== system LunarMicrogrid_Full_Arch/Battery + DAB + Supercap/BESS Controller/DABCtrl2/Ideal P Gain Fdbk ==
  In1 : Inport  SampleTime=SampleTime
  P Gain : Inport  Port=2  SampleTime=SampleTime
  Disabled : Subsystem  VariantControl=Disabled
  External Parameters : Subsystem  VariantControl=ExternalParameters
  Internal Parameters : Subsystem  VariantControl=InternalParameters
  Passthrough : Subsystem  VariantControl=Passthrough
  Out1 : Outport  SampleTime=SampleTime

== system LunarMicrogrid_Full_Arch/Battery + DAB + Supercap/BESS Controller/DABCtrl2/Integrator ==
  U : Inport  SampleTime=SampleTime
  I0in : Inport  Port=2  SampleTime=SampleTime
  Reset : Inport  Port=3  SampleTime=SampleTime
  Continuous : Subsystem  VariantControl=Continuous
  Disabled : Subsystem  VariantControl=Disabled
  Discrete : Subsystem  VariantControl=Discrete
  state : Outport  SampleTime=SampleTime
  out : Outport  Port=2  SampleTime=SampleTime

== system LunarMicrogrid_Full_Arch/Battery + DAB + Supercap/BESS Controller/DABCtrl2/Integrator ICs ==
  I0 : Inport  SampleTime=SampleTime
  Disabled : Subsystem  VariantControl=Disabled
  External IC : Subsystem  VariantControl=ExternalICs
  Internal IC : Subsystem  VariantControl=InternalICs
  Out1 : Outport  SampleTime=SampleTime

== system LunarMicrogrid_Full_Arch/Battery + DAB + Supercap/BESS Controller/DABCtrl2/N Copy ==
  N Gain : Inport  SampleTime=SampleTime
  Disabled : Subsystem  VariantControl=Disabled
  Disabled wSignal Specification : Subsystem  VariantControl=Disabled_SignalSpec
  External Parameters : Subsystem  VariantControl=ExternalParameters
  Internal Parameters : Subsystem  VariantControl=InternalParameters
  Out1 : Outport  SampleTime=SampleTime

== system LunarMicrogrid_Full_Arch/Battery + DAB + Supercap/BESS Controller/DABCtrl2/N Gain ==
  U : Inport  SampleTime=SampleTime
  N Gain : Inport  Port=2  SampleTime=SampleTime
  Disabled : Subsystem  VariantControl=Disabled
  External Parameters : Subsystem  VariantControl=ExternalParameters
  Internal Parameters : Subsystem  VariantControl=InternalParameters
  Passthrough : Subsystem  VariantControl=Passthrough
  Out1 : Outport  SampleTime=SampleTime

== system LunarMicrogrid_Full_Arch/Battery + DAB + Supercap/BESS Controller/DABCtrl2/P Copy ==
  P Gain : Inport  SampleTime=SampleTime
  Disabled : Subsystem  VariantControl=Disabled
  External Parameters Ideal : Subsystem  VariantControl=ExternalParamsIdeal
  Internal Parameters Ideal : Subsystem  VariantControl=InternalParamsIdeal
  Out1 : Outport  SampleTime=SampleTime

== system LunarMicrogrid_Full_Arch/Battery + DAB + Supercap/BESS Controller/DABCtrl2/PID Compensator Formula ==

== system LunarMicrogrid_Full_Arch/Battery + DAB + Supercap/BESS Controller/DABCtrl2/Parallel P Gain ==
  err : Inport  SampleTime=SampleTime
  P Gain : Inport  Port=2  SampleTime=SampleTime
  Disabled : Subsystem  VariantControl=Disabled
  External Parameters : Subsystem  VariantControl=ExternalParameters
  Internal Parameters : Subsystem  VariantControl=InternalParameters
  Passthrough : Subsystem  VariantControl=Passthrough
  Out1 : Outport  SampleTime=SampleTime

== system LunarMicrogrid_Full_Arch/Battery + DAB + Supercap/BESS Controller/DABCtrl2/Reset Signal ==
  Reset : Inport  SampleTime=SampleTime
  Disabled : Subsystem  VariantControl=Disabled
  External Reset : Subsystem  VariantControl=ExternalReset
  Out1 : Outport  SampleTime=SampleTime

== system LunarMicrogrid_Full_Arch/Battery + DAB + Supercap/BESS Controller/DABCtrl2/Saturation ==
  In1 : Inport  SampleTime=SampleTime
  Upper Limit : Inport  Port=2  SampleTime=SampleTime
  Lower Limit : Inport  Port=3  SampleTime=SampleTime
  Enabled : Subsystem  VariantControl=Enabled
  External : Subsystem  VariantControl=External
  Passthrough : Subsystem  VariantControl=Disabled
  Out1 : Outport  SampleTime=SampleTime

== system LunarMicrogrid_Full_Arch/Battery + DAB + Supercap/BESS Controller/DABCtrl2/Saturation Fdbk ==
  In1 : Inport  SampleTime=SampleTime
  Upper Limit : Inport  Port=2  SampleTime=SampleTime
  Lower Limit : Inport  Port=3  SampleTime=SampleTime
  Disabled : Subsystem  VariantControl=Disabled
  Enabled : Subsystem  VariantControl=Enabled
  External : Subsystem  VariantControl=External
  Passthrough : Subsystem  VariantControl=Passthrough
  Out1 : Outport  SampleTime=SampleTime

== system LunarMicrogrid_Full_Arch/Battery + DAB + Supercap/BESS Controller/DABCtrl2/Sum ==
  P : Inport  SampleTime=SampleTime
  I : Inport  Port=2  SampleTime=SampleTime
  D : Inport  Port=3  SampleTime=SampleTime
  Passthrough_I : Subsystem  VariantControl=Passthrough_I
  Passthrough_P : Subsystem  VariantControl=Passthrough_P
  Sum_PD : Subsystem  VariantControl=Sum_PD
  Sum_PI : Subsystem  VariantControl=Sum_PI
  Sum_PID : Subsystem  VariantControl=Sum_PID
  Out1 : Outport  SampleTime=SampleTime

== system LunarMicrogrid_Full_Arch/Battery + DAB + Supercap/BESS Controller/DABCtrl2/Sum Fdbk ==
  fromP : Inport  SampleTime=SampleTime
  fromState : Inport  Port=2  SampleTime=SampleTime
  fromD : Inport  Port=3  SampleTime=SampleTime
  Disabled : Subsystem  VariantControl=Disabled
  Enabled : Subsystem  VariantControl=Enabled
  Passthrough : Subsystem  VariantControl=Passthrough
  Out1 : Outport  SampleTime=SampleTime

== system LunarMicrogrid_Full_Arch/Battery + DAB + Supercap/BESS Controller/DABCtrl2/Tracking Mode ==
  uout : Inport  SampleTime=SampleTime
  TR : Inport  Port=2  SampleTime=SampleTime
  Disabled : Subsystem  VariantControl=Disabled
  Enabled : Subsystem  VariantControl=Enabled
  Out1 : Outport  SampleTime=SampleTime

== system LunarMicrogrid_Full_Arch/Battery + DAB + Supercap/BESS Controller/DABCtrl2/Tracking Mode Sum ==
  fromIgain : Inport  SampleTime=SampleTime
  fromTR : Inport  Port=2  SampleTime=SampleTime
  Passthrough : Subsystem  VariantControl=Passthrough
  Tracking Mode : Subsystem  VariantControl=TrackingMode
  preInt : Outport

== system LunarMicrogrid_Full_Arch/Battery + DAB + Supercap/BESS Controller/DABCtrl2/Tsamp - Integral ==
  U : Inport  SampleTime=SampleTime
  Ts : Inport  Port=2  SampleTime=SampleTime
  Disabled : Subsystem  VariantControl=Disabled
  External Ts : Subsystem  VariantControl=ExternalTs
  Passthrough : Subsystem  VariantControl=Passthrough
  TsSignalSpecification : Subsystem  VariantControl=Disabled_SignalSpec
  Out1 : Outport  SampleTime=SampleTime

== system LunarMicrogrid_Full_Arch/Battery + DAB + Supercap/BESS Controller/DABCtrl2/Tsamp - Ngain ==
  U : Inport  SampleTime=SampleTime
  Ts : Inport  Port=2  SampleTime=SampleTime
  External Ts : Subsystem  VariantControl=ExternalTs
  Passthrough : Subsystem  VariantControl=Passthrough
  Out1 : Outport  SampleTime=SampleTime

== system LunarMicrogrid_Full_Arch/Battery + DAB + Supercap/BESS Controller/DABCtrl2/postSat Signal ==
  feedback : Inport  SampleTime=SampleTime
  forward : Inport  Port=2  SampleTime=SampleTime
  Feedback_Path : Subsystem  VariantControl=Feedback
  Forward_Path : Subsystem  VariantControl=Forward
  Out1 : Outport  SampleTime=SampleTime

== system LunarMicrogrid_Full_Arch/Battery + DAB + Supercap/BESS Controller/DABCtrl2/preInt Signal ==
  preInt : Inport  SampleTime=SampleTime
  extAW : Inport  Port=2  SampleTime=SampleTime
  External PreInt : Subsystem  VariantControl=ExternalPreInt
  Internal PreInt : Subsystem  VariantControl=InternalPreInt
  Out1 : Outport  SampleTime=SampleTime

== system LunarMicrogrid_Full_Arch/Battery + DAB + Supercap/BESS Controller/DABCtrl2/preSat Signal ==
  feedback : Inport  SampleTime=SampleTime
  forward : Inport  Port=2  SampleTime=SampleTime
  Feedback_Path : Subsystem  VariantControl=Feedback
  Forward_Path : Subsystem  VariantControl=Forward
  Out1 : Outport  SampleTime=SampleTime

== system LunarMicrogrid_Full_Arch/Battery + DAB + Supercap/BESS Controller/PIctrl/Anti-windup ==
  preSat : Inport  SampleTime=SampleTime
  postSat : Inport  Port=2  SampleTime=SampleTime
  P : Inport  Port=3  SampleTime=SampleTime
  preInt : Inport  Port=4  SampleTime=SampleTime
  Upper Limit : Inport  Port=5  SampleTime=SampleTime
  Lower Limit : Inport  Port=6  SampleTime=SampleTime
  Back Calculation : Subsystem  VariantControl=BackCalculation
  Cont. Clamping Ideal : Subsystem  VariantControl=ContClampingIdeal
  Cont. Clamping Parallel : Subsystem  VariantControl=ContClampingParallel
  Disabled : Subsystem  VariantControl=Disabled
  Disc. Clamping Ideal : Subsystem  VariantControl=DiscClampingIdeal
  Disc. Clamping Parallel : Subsystem  VariantControl=DiscClampingParallel
  Passthrough : Subsystem  VariantControl=Passthrough
  Out1 : Outport  SampleTime=SampleTime

== system LunarMicrogrid_Full_Arch/Battery + DAB + Supercap/BESS Controller/PIctrl/D Gain ==
  err : Inport  SampleTime=SampleTime
  D Gain : Inport  Port=2  SampleTime=SampleTime
  Disabled : Subsystem  VariantControl=Disabled
  External Parameters : Subsystem  VariantControl=ExternalParameters
  Internal Parameters : Subsystem  VariantControl=InternalParameters
  Out1 : Outport  SampleTime=SampleTime

== system LunarMicrogrid_Full_Arch/Battery + DAB + Supercap/BESS Controller/PIctrl/External Derivative ==
  err : Inport  SampleTime=SampleTime
  ydot : Inport  Port=2  SampleTime=SampleTime
  Disabled : Subsystem  VariantControl=Disabled
  Error : Subsystem  VariantControl=ErrorSignal
  External Ydot : Subsystem  VariantControl=ExternalYdot
  Out1 : Outport  SampleTime=SampleTime

== system LunarMicrogrid_Full_Arch/Battery + DAB + Supercap/BESS Controller/PIctrl/Filter ==
  Reset : Inport  SampleTime=SampleTime
  U : Inport  Port=2  SampleTime=SampleTime
  N : Inport  Port=3  SampleTime=SampleTime
  D0in : Inport  Port=4  SampleTime=SampleTime
  Nout : Inport  Port=5  SampleTime=SampleTime
  Ts : Inport  Port=6  SampleTime=SampleTime
  Cont. Filter : Subsystem  VariantControl=ContFilter
  Cont. Filter Only : Subsystem  VariantControl=ContFilterOnly
  Differentiator : Subsystem  VariantControl=Differentiator
  Disabled : Subsystem  VariantControl=Disabled
  Disc. Backward Euler Filter : Subsystem  VariantControl=BackwardEulerFilter
  Disc. Backward Euler Filter Only : Subsystem  VariantControl=BackwardEulerFilterOnly
  Disc. Forward Euler Filter : Subsystem  VariantControl=ForwardEulerFilter
  Disc. Forward Euler Filter Only : Subsystem  VariantControl=ForwardEulerFilterOnly
  Disc. Trapezoidal Filter : Subsystem  VariantControl=TrapezoidalFilter
  Disc. Trapezoidal Filter Only : Subsystem  VariantControl=TrapezoidalFilterOnly
  Passthrough : Subsystem  VariantControl=Passthrough
  Y : Outport  SampleTime=SampleTime

== system LunarMicrogrid_Full_Arch/Battery + DAB + Supercap/BESS Controller/PIctrl/Filter ICs ==
  D0 : Inport  SampleTime=SampleTime
  Disabled : Subsystem  VariantControl=Disabled
  External IC : Subsystem  VariantControl=ExternalICs
  Internal IC - Differentiator : Subsystem  VariantControl=InternalICsDifferentiator
  Internal IC - Filter : Subsystem  VariantControl=InternalICsFilter
  Out1 : Outport  SampleTime=SampleTime

== system LunarMicrogrid_Full_Arch/Battery + DAB + Supercap/BESS Controller/PIctrl/I Gain ==
  err : Inport  SampleTime=SampleTime
  I Gain : Inport  Port=2  SampleTime=SampleTime
  Disabled : Subsystem  VariantControl=Disabled
  External Parameters : Subsystem  VariantControl=ExternalParameters
  Internal Parameters : Subsystem  VariantControl=InternalParameters
  Out1 : Outport  SampleTime=SampleTime

== system LunarMicrogrid_Full_Arch/Battery + DAB + Supercap/BESS Controller/PIctrl/Ideal P Gain ==
  In1 : Inport  SampleTime=SampleTime
  P Gain : Inport  Port=2  SampleTime=SampleTime
  External Parameters : Subsystem  VariantControl=ExternalParameters
  Internal Parameters : Subsystem  VariantControl=InternalParameters
  Passthrough : Subsystem  VariantControl=Disabled
  Out1 : Outport  SampleTime=SampleTime

== system LunarMicrogrid_Full_Arch/Battery + DAB + Supercap/BESS Controller/PIctrl/Ideal P Gain Fdbk ==
  In1 : Inport  SampleTime=SampleTime
  P Gain : Inport  Port=2  SampleTime=SampleTime
  Disabled : Subsystem  VariantControl=Disabled
  External Parameters : Subsystem  VariantControl=ExternalParameters
  Internal Parameters : Subsystem  VariantControl=InternalParameters
  Passthrough : Subsystem  VariantControl=Passthrough
  Out1 : Outport  SampleTime=SampleTime

== system LunarMicrogrid_Full_Arch/Battery + DAB + Supercap/BESS Controller/PIctrl/Integrator ==
  U : Inport  SampleTime=SampleTime
  I0in : Inport  Port=2  SampleTime=SampleTime
  Reset : Inport  Port=3  SampleTime=SampleTime
  Continuous : Subsystem  VariantControl=Continuous
  Disabled : Subsystem  VariantControl=Disabled
  Discrete : Subsystem  VariantControl=Discrete
  state : Outport  SampleTime=SampleTime
  out : Outport  Port=2  SampleTime=SampleTime

== system LunarMicrogrid_Full_Arch/Battery + DAB + Supercap/BESS Controller/PIctrl/Integrator ICs ==
  I0 : Inport  SampleTime=SampleTime
  Disabled : Subsystem  VariantControl=Disabled
  External IC : Subsystem  VariantControl=ExternalICs
  Internal IC : Subsystem  VariantControl=InternalICs
  Out1 : Outport  SampleTime=SampleTime

== system LunarMicrogrid_Full_Arch/Battery + DAB + Supercap/BESS Controller/PIctrl/N Copy ==
  N Gain : Inport  SampleTime=SampleTime
  Disabled : Subsystem  VariantControl=Disabled
  Disabled wSignal Specification : Subsystem  VariantControl=Disabled_SignalSpec
  External Parameters : Subsystem  VariantControl=ExternalParameters
  Internal Parameters : Subsystem  VariantControl=InternalParameters
  Out1 : Outport  SampleTime=SampleTime
